simulink model "LineFollower_8Sensors_P"  (R2024b)
settings: Solver=ode45  StartTime=0.0  StopTime=10  MaxStep=0.005  RelTol=1e-3
model workspace (MAT data in the model file):
  Kp = 5
  baseSpeed = 0.08
  errorGain = 0.001
  wheelBase = 0.15
  wheelRadius = 0.033
settings Model: Creator=Devansh  LastModifiedBy=Devansh

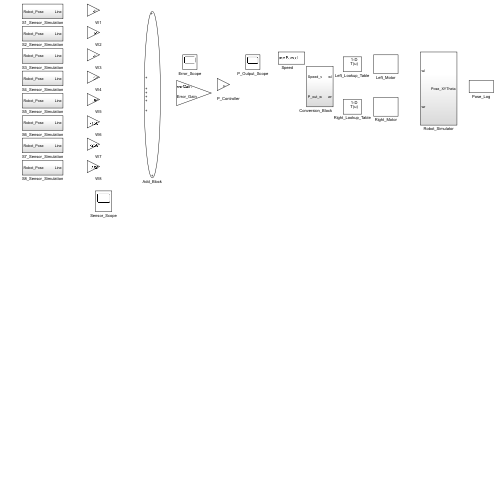
[thumbnail: Simulink's stored preview of the top-level diagram]
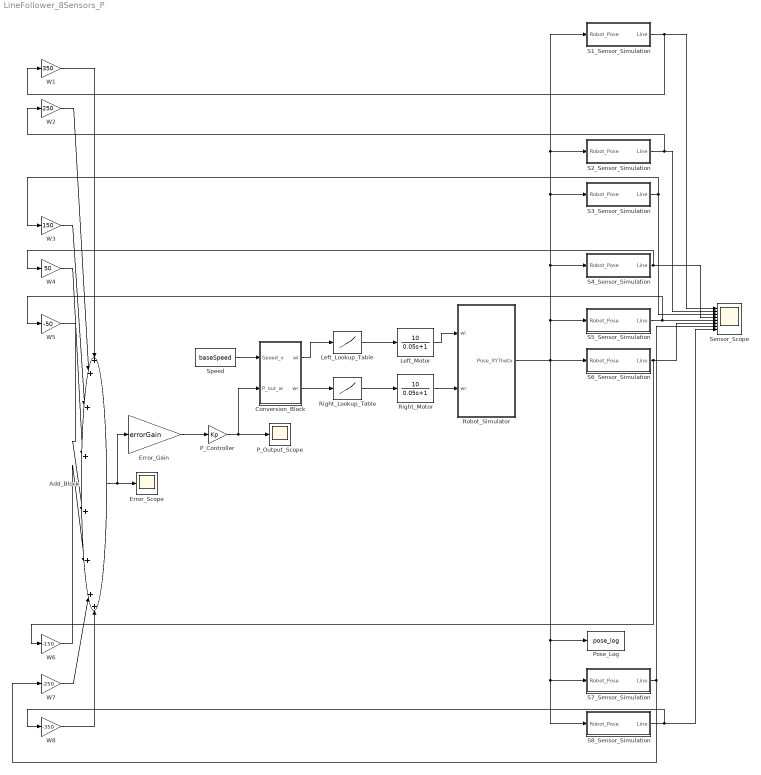
== system LineFollower_8Sensors_P ==
  Add_Block : Sum  Inputs=++++++++
  Conversion_Block : Subsystem
  Error_Gain : Gain  Gain=errorGain
  Error_Scope : Scope
  Left_Lookup_Table : Lookup_n-D  NumberOfTableDimensions=1  BreakpointsForDimension1=[-1 0 1]  Table=[-1 0 1]  InternalRulePriority=Speed  RndMeth=Simplest
  Left_Motor : TransferFcn  Numerator=[10]  Denominator=[0.05 1]
  P_Controller : Gain  Gain=Kp
  P_Output_Scope : Scope
  Pose_Log : ToWorkspace  VariableName=pose_log  SampleTime=-1
  Right_Lookup_Table : Lookup_n-D  NumberOfTableDimensions=1  BreakpointsForDimension1=[-1 0 1]  Table=[-1 0 1]  InternalRulePriority=Speed  RndMeth=Simplest
  Right_Motor : TransferFcn  Numerator=[10]  Denominator=[0.05 1]
  Robot_Simulator : Subsystem
  S1_Sensor_Simulation : Subsystem
  S2_Sensor_Simulation : Subsystem
  S3_Sensor_Simulation : Subsystem
  S4_Sensor_Simulation : Subsystem
  S5_Sensor_Simulation : Subsystem
  S6_Sensor_Simulation : Subsystem
  S7_Sensor_Simulation : Subsystem
  S8_Sensor_Simulation : Subsystem
  Sensor_Scope : Scope  NumInputPorts=8
  Speed : Constant  Value=baseSpeed
  W1 : Gain  Gain=350
  W2 : Gain  Gain=250
  W3 : Gain  Gain=150
  W4 : Gain  Gain=50
  W5 : Gain  Gain=-50
  W6 : Gain  Gain=-150
  W7 : Gain  Gain=-250
  W8 : Gain  Gain=-350
  wires:
  W5/1 -> Add_Block/5
  S1_Sensor_Simulation/1(Line) -> W1/1, Sensor_Scope/1
  W1/1 -> Add_Block/1
  S2_Sensor_Simulation/1(Line) -> Sensor_Scope/2, W2/1
  W7/1 -> Add_Block/7
  W2/1 -> Add_Block/2
  P_Controller/1 -> Conversion_Block/2(P_out_w), P_Output_Scope/1
  W3/1 -> Add_Block/3
  W4/1 -> Add_Block/4
  Robot_Simulator/1(Pose_XYTheta) -> S7_Sensor_Simulation/1(Robot_Pose), S8_Sensor_Simulation/1(Robot_Pose), Pose_Log/1, S1_Sensor_Simulation/1(Robot_Pose), S2_Sensor_Simulation/1(Robot_Pose), S3_Sensor_Simulation/1(Robot_Pose), S4_Sensor_Simulation/1(Robot_Pose), S5_Sensor_Simulation/1(Robot_Pose), S6_Sensor_Simulation/1(Robot_Pose)
  W6/1 -> Add_Block/6
  Left_Lookup_Table/1 -> Left_Motor/1
  W8/1 -> Add_Block/8
  Add_Block/1 -> Error_Gain/1, Error_Scope/1
  Error_Gain/1 -> P_Controller/1
  Speed/1 -> Conversion_Block/1(Speed_v)
  Conversion_Block/1(wl) -> Left_Lookup_Table/1
  Conversion_Block/2(wr) -> Right_Lookup_Table/1
  Right_Lookup_Table/1 -> Right_Motor/1
  Right_Motor/1 -> Robot_Simulator/2(wr)
  Left_Motor/1 -> Robot_Simulator/1(wl)
  S3_Sensor_Simulation/1(Line) -> W3/1, Sensor_Scope/3
  S4_Sensor_Simulation/1(Line) -> W4/1, Sensor_Scope/4
  S5_Sensor_Simulation/1(Line) -> W5/1, Sensor_Scope/5
  S6_Sensor_Simulation/1(Line) -> W6/1, Sensor_Scope/6
  S7_Sensor_Simulation/1(Line) -> W7/1, Sensor_Scope/7
  S8_Sensor_Simulation/1(Line) -> W8/1, Sensor_Scope/8

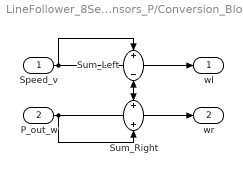
== system LineFollower_8Sensors_P/Conversion_Block ==
  Speed_v : Inport
  P_out_w : Inport  Port=2
  Sum_Left : Sum  Inputs=+-
  Sum_Right : Sum
  wl : Outport
  wr : Outport  Port=2
  wires:
  Speed_v/1 -> Sum_Left/1, Sum_Right/1
  P_out_w/1 -> Sum_Left/2, Sum_Right/2
  Sum_Left/1 -> wl/1
  Sum_Right/1 -> wr/1

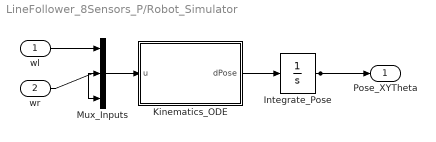
== system LineFollower_8Sensors_P/Robot_Simulator ==
  wl : Inport
  wr : Inport  Port=2
  Integrate_Pose : Integrator  InitialCondition=[0; 0; 0]
  Kinematics_ODE : MATLAB Function  TreatAsAtomicUnit=on
  Mux_Inputs : Mux  Inputs=3
  Pose_XYTheta : Outport
  wires:
  wl/1 -> Mux_Inputs/1
  wr/1 -> Mux_Inputs/2
  Integrate_Pose/1 -> Mux_Inputs/3, Pose_XYTheta/1
  Mux_Inputs/1 -> Kinematics_ODE/1(u)
  Kinematics_ODE/1(dPose) -> Integrate_Pose/1

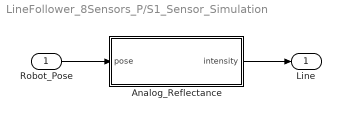
== system LineFollower_8Sensors_P/S1_Sensor_Simulation ==
  Robot_Pose : Inport
  Analog_Reflectance : MATLAB Function  TreatAsAtomicUnit=on
  Line : Outport
  wires:
  Robot_Pose/1 -> Analog_Reflectance/1(pose)
  Analog_Reflectance/1(intensity) -> Line/1

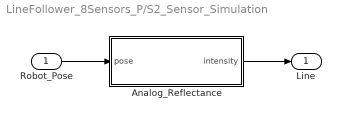
== system LineFollower_8Sensors_P/S2_Sensor_Simulation ==
  Robot_Pose : Inport
  Analog_Reflectance : MATLAB Function  TreatAsAtomicUnit=on
  Line : Outport
  wires:
  Robot_Pose/1 -> Analog_Reflectance/1(pose)
  Analog_Reflectance/1(intensity) -> Line/1

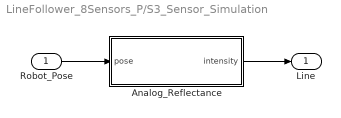
== system LineFollower_8Sensors_P/S3_Sensor_Simulation ==
  Robot_Pose : Inport
  Analog_Reflectance : MATLAB Function  TreatAsAtomicUnit=on
  Line : Outport
  wires:
  Robot_Pose/1 -> Analog_Reflectance/1(pose)
  Analog_Reflectance/1(intensity) -> Line/1

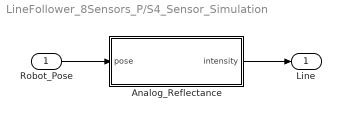
== system LineFollower_8Sensors_P/S4_Sensor_Simulation ==
  Robot_Pose : Inport
  Analog_Reflectance : MATLAB Function  TreatAsAtomicUnit=on
  Line : Outport
  wires:
  Robot_Pose/1 -> Analog_Reflectance/1(pose)
  Analog_Reflectance/1(intensity) -> Line/1

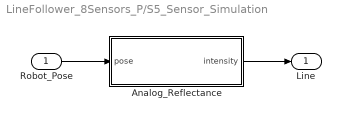
== system LineFollower_8Sensors_P/S5_Sensor_Simulation ==
  Robot_Pose : Inport
  Analog_Reflectance : MATLAB Function  TreatAsAtomicUnit=on
  Line : Outport
  wires:
  Robot_Pose/1 -> Analog_Reflectance/1(pose)
  Analog_Reflectance/1(intensity) -> Line/1

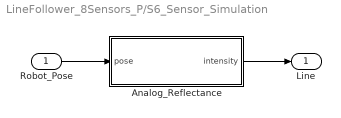
== system LineFollower_8Sensors_P/S6_Sensor_Simulation ==
  Robot_Pose : Inport
  Analog_Reflectance : MATLAB Function  TreatAsAtomicUnit=on
  Line : Outport
  wires:
  Robot_Pose/1 -> Analog_Reflectance/1(pose)
  Analog_Reflectance/1(intensity) -> Line/1

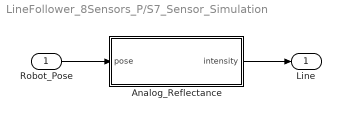
== system LineFollower_8Sensors_P/S7_Sensor_Simulation ==
  Robot_Pose : Inport
  Analog_Reflectance : MATLAB Function  TreatAsAtomicUnit=on
  Line : Outport
  wires:
  Robot_Pose/1 -> Analog_Reflectance/1(pose)
  Analog_Reflectance/1(intensity) -> Line/1

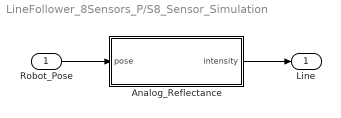
== system LineFollower_8Sensors_P/S8_Sensor_Simulation ==
  Robot_Pose : Inport
  Analog_Reflectance : MATLAB Function  TreatAsAtomicUnit=on
  Line : Outport
  wires:
  Robot_Pose/1 -> Analog_Reflectance/1(pose)
  Analog_Reflectance/1(intensity) -> Line/1

== matlab function LineFollower_8Sensors_P/S1_Sensor_Simulation/Analog_Reflectance ==
  data: pose input; intensity output
function intensity = Analog_Reflectance(pose)
% Continuous optical Gaussian reflectance
x = pose(1);
y = pose(2);
theta = pose(3);
pitch = 0.009; % 9mm spacing
d_offset = (-3.500000) * pitch;
forward_offset = 0.06;
sx = x + forward_offset*cos(theta) - d_offset*sin(theta);
sy = y + forward_offset*sin(theta) + d_offset*cos(theta);
y_line = 0.05 * sin(2*pi*sx / 2.0);
dist = abs(sy - y_line);
sigma = 0.012;
intensity = exp(- (dist^2) / (2 * sigma^2)); % Continuous [0, 1]
end

== matlab function LineFollower_8Sensors_P/S3_Sensor_Simulation/Analog_Reflectance ==
  data: pose input; intensity output
function intensity = Analog_Reflectance(pose)
% Continuous optical Gaussian reflectance
x = pose(1);
y = pose(2);
theta = pose(3);
pitch = 0.009; % 9mm spacing
d_offset = (-1.500000) * pitch;
forward_offset = 0.06;
sx = x + forward_offset*cos(theta) - d_offset*sin(theta);
sy = y + forward_offset*sin(theta) + d_offset*cos(theta);
y_line = 0.05 * sin(2*pi*sx / 2.0);
dist = abs(sy - y_line);
sigma = 0.012;
intensity = exp(- (dist^2) / (2 * sigma^2)); % Continuous [0, 1]
end

== matlab function LineFollower_8Sensors_P/S4_Sensor_Simulation/Analog_Reflectance ==
  data: pose input; intensity output
function intensity = Analog_Reflectance(pose)
% Continuous optical Gaussian reflectance
x = pose(1);
y = pose(2);
theta = pose(3);
pitch = 0.009; % 9mm spacing
d_offset = (-0.500000) * pitch;
forward_offset = 0.06;
sx = x + forward_offset*cos(theta) - d_offset*sin(theta);
sy = y + forward_offset*sin(theta) + d_offset*cos(theta);
y_line = 0.05 * sin(2*pi*sx / 2.0);
dist = abs(sy - y_line);
sigma = 0.012;
intensity = exp(- (dist^2) / (2 * sigma^2)); % Continuous [0, 1]
end

== matlab function LineFollower_8Sensors_P/S5_Sensor_Simulation/Analog_Reflectance ==
  data: pose input; intensity output
function intensity = Analog_Reflectance(pose)
% Continuous optical Gaussian reflectance
x = pose(1);
y = pose(2);
theta = pose(3);
pitch = 0.009; % 9mm spacing
d_offset = (0.500000) * pitch;
forward_offset = 0.06;
sx = x + forward_offset*cos(theta) - d_offset*sin(theta);
sy = y + forward_offset*sin(theta) + d_offset*cos(theta);
y_line = 0.05 * sin(2*pi*sx / 2.0);
dist = abs(sy - y_line);
sigma = 0.012;
intensity = exp(- (dist^2) / (2 * sigma^2)); % Continuous [0, 1]
end

== matlab function LineFollower_8Sensors_P/S6_Sensor_Simulation/Analog_Reflectance ==
  data: pose input; intensity output
function intensity = Analog_Reflectance(pose)
% Continuous optical Gaussian reflectance
x = pose(1);
y = pose(2);
theta = pose(3);
pitch = 0.009; % 9mm spacing
d_offset = (1.500000) * pitch;
forward_offset = 0.06;
sx = x + forward_offset*cos(theta) - d_offset*sin(theta);
sy = y + forward_offset*sin(theta) + d_offset*cos(theta);
y_line = 0.05 * sin(2*pi*sx / 2.0);
dist = abs(sy - y_line);
sigma = 0.012;
intensity = exp(- (dist^2) / (2 * sigma^2)); % Continuous [0, 1]
end

== matlab function LineFollower_8Sensors_P/S7_Sensor_Simulation/Analog_Reflectance ==
  data: pose input; intensity output
function intensity = Analog_Reflectance(pose)
% Continuous optical Gaussian reflectance
x = pose(1);
y = pose(2);
theta = pose(3);
pitch = 0.009; % 9mm spacing
d_offset = (2.500000) * pitch;
forward_offset = 0.06;
sx = x + forward_offset*cos(theta) - d_offset*sin(theta);
sy = y + forward_offset*sin(theta) + d_offset*cos(theta);
y_line = 0.05 * sin(2*pi*sx / 2.0);
dist = abs(sy - y_line);
sigma = 0.012;
intensity = exp(- (dist^2) / (2 * sigma^2)); % Continuous [0, 1]
end

== matlab function LineFollower_8Sensors_P/S8_Sensor_Simulation/Analog_Reflectance ==
  data: pose input; intensity output
function intensity = Analog_Reflectance(pose)
% Continuous optical Gaussian reflectance
x = pose(1);
y = pose(2);
theta = pose(3);
pitch = 0.009; % 9mm spacing
d_offset = (3.500000) * pitch;
forward_offset = 0.06;
sx = x + forward_offset*cos(theta) - d_offset*sin(theta);
sy = y + forward_offset*sin(theta) + d_offset*cos(theta);
y_line = 0.05 * sin(2*pi*sx / 2.0);
dist = abs(sy - y_line);
sigma = 0.012;
intensity = exp(- (dist^2) / (2 * sigma^2)); % Continuous [0, 1]
end

== matlab function LineFollower_8Sensors_P/Robot_Simulator/Kinematics_ODE ==
  data: u input; dPose output
function dPose = Kinematics_ODE(u)
% u = [wl; wr; x; y; theta]
wl    = u(1);
wr    = u(2);
theta = u(5);
R = 0.033;
L = 0.150;
v = (R/2) * (wr + wl);
omega = (R/L) * (wr - wl);
dPose = [v * cos(theta); v * sin(theta); omega];
end

== matlab function LineFollower_8Sensors_P/S2_Sensor_Simulation/Analog_Reflectance ==
  data: pose input; intensity output
function intensity = Analog_Reflectance(pose)
% Continuous optical Gaussian reflectance
x = pose(1);
y = pose(2);
theta = pose(3);
pitch = 0.009; % 9mm spacing
d_offset = (-2.500000) * pitch;
forward_offset = 0.06;
sx = x + forward_offset*cos(theta) - d_offset*sin(theta);
sy = y + forward_offset*sin(theta) + d_offset*cos(theta);
y_line = 0.05 * sin(2*pi*sx / 2.0);
dist = abs(sy - y_line);
sigma = 0.012;
intensity = exp(- (dist^2) / (2 * sigma^2)); % Continuous [0, 1]
end
